simulink library "ConverterLibrary"  (R2026a)
settings: Solver=VariableStepAuto
undefined symbols (not defined in the file or in its folder): DiscIntNeverNeededParam, dspblkCoreblockFVToolHelper, gcbh, gridInverter
libraries: fl_lib x240, nesl_utility x221, ee_lib x208, slpidlib x28, eeGeneralControl x12, simulink x9, eeTransforms x4, simulink_extras x1, eePowerMeasurement x1
(part 9 of 30)

== system ConverterLibrary/Power Converter Plant/Non-Isolated DC-DC Converters/Non-Isolated DC-DC Converter/NonIsolatedDCDCVariant/Boost ==
  G : Inport
  Co : ee_lib/Passive/Capacitor  cap_option=ee.enum.passive.capacitor.capOption.const  c=C_SI F  Cvec=[1e-05, 1e-06] F  Vvec=[0, 10] V  CV_table_symmetry=ee.enum.passive.capacitor.tableSymmetry.yes  f_vec=[1, 10] kHz  DFext_vec=[.8, 1.2]  enable_C_tol=ee.enum.toleranceApplication.none  averaging_period=0 s  C_tol=5  tol_distribution=ee.enum.toleranceDistribution.uniform  nSigma=4  r=Rco_SI Ohm  g=1e-05 1/Ohm  enable_operating_limits=ee.enum.enable.no  operating_limit_action=ee.enum.passive.reportOpLim.warn  max_working_voltage_range=[-25, 25] V  power_rating=1 W  maxTemperature=85 degC  thermalEnable=false  thermalMass=1 J/K  i_specify=off  i_priority=None  i=0 A  i_nominal_specify=off  i_nominal_value=1  i_nominal_unit=A  v_specify=off  v_priority=None  v=0 V  v_nominal_specify=off  v_nominal_value=1  v_nominal_unit=V  vc_specify=on  vc_priority=High  vc=Vco_SI V  vc_nominal_specify=off  vc_nominal_value=1  vc_nominal_unit=V  T_specify=off  T_priority=None  T=298.15 K  T_nominal_specify=off  T_nominal_value=1  T_nominal_unit=K
  Diode : Subsystem  Variant=on  VariantControlMode=label  LabelModeActiveChoice=IdealDiode
  IL : Subsystem
      mask Display: disp('I')
  Iout : Subsystem
      mask Display: disp('I')
  Lin : ee_lib/Passive/Inductor  l=L_SI H  enable_L_tol=ee.enum.toleranceApplication.none  L_tol=20  tol_distribution=ee.enum.toleranceDistribution.uniform  nSigma=4  r=RL_SI Ohm  g=1e-05 1/Ohm  enable_operating_limits=ee.enum.enable.no  operating_limit_action=ee.enum.passive.reportOpLim.warn  max_working_current=1 A  power_rating=1 W  i_L_specify=off  i_L_priority=High  i_L=0 A  i_L_nominal_specify=off  i_L_nominal_value=1  i_L_nominal_unit=A
  MainSwitch : Subsystem  Variant=on  VariantControlMode=label  LabelModeActiveChoice=IdealSwitch
  Vin : Subsystem
      mask Display: disp('V')
  Vout : Subsystem
      settings: PortSchema="{\"entries\":[{\"content\":{\"sides\":[{\"content\":{\"connectorIds\":[\"LConn1\"]},\"type\":\"ConnectorPlacement.EquallySpacedRectSide\",\"uuid\":\"5f92137b-4b58-46b8-a68f-d3527484291c\"},{\"content\":{\"connectorIds\":[\"RConn1\",\"Out1\"],\"side\":\"RIGHT\"},\"type\":\"ConnectorPlacement.EquallySpacedRectSide\",\"uuid\":\"154b36f0-aa4a-4375-80c2-9c55af429c32\"},{\"content\":{\"side\":\"TOP\"},\"type\":\"ConnectorPlacement.EquallySpacedRectSide\",\"uuid\":\"6e01dd2b-817e-4c7e-a9bf-e017a248a3a8\"}]},\"type\":\"ConnectorPlacement.EquallySpacedConnector\",\"uuid\":\"a9d15cc4-68aa-466b-9599-7a273210f999\"}],\"packageUris\":[\"http://schema.mathworks.com/mf0/Connector/R2020b\"],\"version\":\"1.0\"}"
      mask Display: disp('V')
  Vin+ : PMIOPort  Side=Left
  Vin- : PMIOPort  Port=2  Side=Left
  Vout+ : PMIOPort  Port=3  Side=Right
  Vout- : PMIOPort  Port=4  Side=Right
  Out Bus Element1 : Outport  PortName=meas  Element=IL [A]
  Out Bus Element2 : Outport  PortName=meas  Element=Vout [V]
  Out Bus Element3 : Outport  PortName=meas  Element=Iin [A]
  Out Bus Element4 : Outport  PortName=meas  Element=Vin [V]
  Out Bus Element5 : Outport  PortName=meas  Element=Iout [A]
  wires:
  G/1 -> MainSwitch/1(G)
  Iout/1(I) -> Out Bus Element5/1
  Vin/1(V) -> Out Bus Element4/1
  IL/1(I) -> Out Bus Element3/1, Out Bus Element1/1
  Vout/1(V) -> Out Bus Element2/1
  connections:
  Iout/LConn1 -- Co/LConn1 -- Diode/RConn1
  Diode/LConn1 -- MainSwitch/LConn1 -- Lin/RConn1
  Vin/RConn1 -- Vin-/RConn1 -- Vout/RConn1 -- Vout-/RConn1 -- Co/RConn1 -- MainSwitch/RConn1
  Vout/LConn1 -- Iout/RConn1 -- Vout+/RConn1
  IL/RConn1 -- Lin/LConn1
  IL/LConn1 -- Vin/LConn1 -- Vin+/RConn1

== system ConverterLibrary/Power Converter Plant/Non-Isolated DC-DC Converters/Non-Isolated DC-DC Converter/NonIsolatedDCDCVariant/Buck ==
  G : Inport
  Co : ee_lib/Passive/Capacitor  cap_option=ee.enum.passive.capacitor.capOption.const  c=C_SI F  Cvec=[1e-05, 1e-06] F  Vvec=[0, 10] V  CV_table_symmetry=ee.enum.passive.capacitor.tableSymmetry.yes  f_vec=[1, 10] kHz  DFext_vec=[.8, 1.2]  enable_C_tol=ee.enum.toleranceApplication.none  averaging_period=0 s  C_tol=5  tol_distribution=ee.enum.toleranceDistribution.uniform  nSigma=4  r=Rco_SI Ohm  g=1e-05 1/Ohm  enable_operating_limits=ee.enum.enable.no  operating_limit_action=ee.enum.passive.reportOpLim.warn  max_working_voltage_range=[-25, 25] V  power_rating=1 W  maxTemperature=85 degC  thermalEnable=false  thermalMass=1 J/K  i_specify=off  i_priority=None  i=0 A  i_nominal_specify=off  i_nominal_value=1  i_nominal_unit=A  v_specify=off  v_priority=None  v=0 V  v_nominal_specify=off  v_nominal_value=1  v_nominal_unit=V  vc_specify=on  vc_priority=High  vc=Vco_SI V  vc_nominal_specify=off  vc_nominal_value=1  vc_nominal_unit=V  T_specify=off  T_priority=None  T=298.15 K  T_nominal_specify=off  T_nominal_value=1  T_nominal_unit=K
  Diode : Subsystem  Variant=on  VariantControlMode=label  LabelModeActiveChoice=IdealDiode
  IL : Subsystem
      mask Display: disp('I')
  Iin : Subsystem
      mask Display: disp('I')
  Iout : Subsystem
      mask Display: disp('I')
  Lout : ee_lib/Passive/Inductor  l=L_SI H  enable_L_tol=ee.enum.toleranceApplication.none  L_tol=20  tol_distribution=ee.enum.toleranceDistribution.uniform  nSigma=4  r=RL_SI Ohm  g=1e-05 1/Ohm  enable_operating_limits=ee.enum.enable.no  operating_limit_action=ee.enum.passive.reportOpLim.warn  max_working_current=1 A  power_rating=1 W  i_L_specify=off  i_L_priority=High  i_L=0 A  i_L_nominal_specify=off  i_L_nominal_value=1  i_L_nominal_unit=A
  MainSwitch : Subsystem  Variant=on  VariantControlMode=label  LabelModeActiveChoice=IdealSwitch
  Vin : Subsystem
      mask Display: disp('V')
  Vout : Subsystem
      settings: PortSchema="{\"entries\":[{\"content\":{\"sides\":[{\"content\":{\"connectorIds\":[\"LConn1\"]},\"type\":\"ConnectorPlacement.EquallySpacedRectSide\",\"uuid\":\"5f92137b-4b58-46b8-a68f-d3527484291c\"},{\"content\":{\"connectorIds\":[\"RConn1\",\"Out1\"],\"side\":\"RIGHT\"},\"type\":\"ConnectorPlacement.EquallySpacedRectSide\",\"uuid\":\"154b36f0-aa4a-4375-80c2-9c55af429c32\"},{\"content\":{\"side\":\"TOP\"},\"type\":\"ConnectorPlacement.EquallySpacedRectSide\",\"uuid\":\"6e01dd2b-817e-4c7e-a9bf-e017a248a3a8\"}]},\"type\":\"ConnectorPlacement.EquallySpacedConnector\",\"uuid\":\"a9d15cc4-68aa-466b-9599-7a273210f999\"}],\"packageUris\":[\"http://schema.mathworks.com/mf0/Connector/R2020b\"],\"version\":\"1.0\"}"
      mask Display: disp('V')
  Vin+ : PMIOPort  Side=Left
  Vin- : PMIOPort  Port=2  Side=Left
  Vout+ : PMIOPort  Port=3  Side=Right
  Vout- : PMIOPort  Port=4  Side=Right
  Out Bus Element1 : Outport  PortName=meas  Element=IL [A]
  Out Bus Element2 : Outport  PortName=meas  Element=Vout [V]
  Out Bus Element3 : Outport  PortName=meas  Element=Iin [A]
  Out Bus Element4 : Outport  PortName=meas  Element=Vin [V]
  Out Bus Element5 : Outport  PortName=meas  Element=Iout [A]
  wires:
  G/1 -> MainSwitch/1(G)
  Iout/1(I) -> Out Bus Element5/1
  Vin/1(V) -> Out Bus Element4/1
  Iin/1(I) -> Out Bus Element3/1
  Vout/1(V) -> Out Bus Element2/1
  IL/1(I) -> Out Bus Element1/1
  connections:
  Co/RConn1 -- Diode/LConn1 -- Vin/RConn1 -- Vin-/RConn1 -- Vout/RConn1 -- Vout-/RConn1
  Vout/LConn1 -- Vout+/RConn1 -- Iout/RConn1
  Co/LConn1 -- Iout/LConn1 -- IL/RConn1
  Lout/RConn1 -- IL/LConn1
  MainSwitch/RConn1 -- Lout/LConn1 -- Diode/RConn1
  Iin/RConn1 -- MainSwitch/LConn1
  Vin/LConn1 -- Vin+/RConn1 -- Iin/LConn1

== system ConverterLibrary/Power Converter Plant/Non-Isolated DC-DC Converters/Non-Isolated DC-DC Converter/NonIsolatedDCDCVariant/BuckBoost ==
  G : Inport
  Co : ee_lib/Passive/Capacitor  cap_option=ee.enum.passive.capacitor.capOption.const  c=C_SI F  Cvec=[1e-05, 1e-06] F  Vvec=[0, 10] V  CV_table_symmetry=ee.enum.passive.capacitor.tableSymmetry.yes  f_vec=[1, 10] kHz  DFext_vec=[.8, 1.2]  enable_C_tol=ee.enum.toleranceApplication.none  averaging_period=0 s  C_tol=5  tol_distribution=ee.enum.toleranceDistribution.uniform  nSigma=4  r=Rco_SI Ohm  g=1e-05 1/Ohm  enable_operating_limits=ee.enum.enable.no  operating_limit_action=ee.enum.passive.reportOpLim.warn  max_working_voltage_range=[-25, 25] V  power_rating=1 W  maxTemperature=85 degC  thermalEnable=false  thermalMass=1 J/K  i_specify=off  i_priority=None  i=0 A  i_nominal_specify=off  i_nominal_value=1  i_nominal_unit=A  v_specify=off  v_priority=None  v=0 V  v_nominal_specify=off  v_nominal_value=1  v_nominal_unit=V  vc_specify=on  vc_priority=High  vc=Vco_SI V  vc_nominal_specify=off  vc_nominal_value=1  vc_nominal_unit=V  T_specify=off  T_priority=None  T=298.15 K  T_nominal_specify=off  T_nominal_value=1  T_nominal_unit=K
  Diode : Subsystem  Variant=on  VariantControlMode=label  LabelModeActiveChoice=IdealDiode
  IL : Subsystem
      settings: PortSchema="{\"entries\":[{\"content\":{\"sides\":[{\"content\":{\"connectorIds\":[\"LConn1\"]},\"type\":\"ConnectorPlacement.EquallySpacedRectSide\",\"uuid\":\"5f92137b-4b58-46b8-a68f-d3527484291c\"},{\"content\":{\"connectorIds\":[\"RConn1\",\"Out1\"],\"side\":\"RIGHT\"},\"type\":\"ConnectorPlacement.EquallySpacedRectSide\",\"uuid\":\"154b36f0-aa4a-4375-80c2-9c55af429c32\"},{\"content\":{\"side\":\"TOP\"},\"type\":\"ConnectorPlacement.EquallySpacedRectSide\",\"uuid\":\"6e01dd2b-817e-4c7e-a9bf-e017a248a3a8\"},{\"content\":{\"side\":\"BOTTOM\"},\"type\":\"ConnectorPlacement.EquallySpacedRectSide\",\"uuid\":\"8c02900b-7040-4e1d-af3e-df4ce1eee484\"}]},\"type\":\"ConnectorPlacement.EquallySpacedConnector\",\"uuid\":\"a9d15cc4-68aa-466b-9599-7a273210f999\"}],\"packageUris\":[\"http://schema.mathworks.com/mf0/Connector/R2020b\"],\"version\":\"1.0\"}"
      mask Display: disp('I')
  Iin : Subsystem
      mask Display: disp('I')
  Iout : Subsystem
      settings: PortSchema="{\"entries\":[{\"content\":{\"sides\":[{\"content\":{\"connectorIds\":[\"LConn1\"]},\"type\":\"ConnectorPlacement.EquallySpacedRectSide\",\"uuid\":\"7ec392cc-277f-44b1-b35e-7f2730db0397\"},{\"content\":{\"connectorIds\":[\"RConn1\",\"Out1\"],\"side\":\"RIGHT\"},\"type\":\"ConnectorPlacement.EquallySpacedRectSide\",\"uuid\":\"b0b5f2e0-1c59-4384-a465-885626d66149\"},{\"content\":{\"side\":\"TOP\"},\"type\":\"ConnectorPlacement.EquallySpacedRectSide\",\"uuid\":\"04ca4100-95ca-4157-98b9-4ff919847b2d\"}]},\"type\":\"ConnectorPlacement.EquallySpacedConnector\",\"uuid\":\"4f5cd1ed-b6ae-4123-b76e-0cf834717a23\"}],\"packageUris\":[\"http://schema.mathworks.com/mf0/Connector/R2020b\"],\"version\":\"1.0\"}"
      mask Display: disp('I')
  Lstore : ee_lib/Passive/Inductor  l=L_SI H  enable_L_tol=ee.enum.toleranceApplication.none  L_tol=20  tol_distribution=ee.enum.toleranceDistribution.uniform  nSigma=4  r=RL_SI Ohm  g=1e-05 1/Ohm  enable_operating_limits=ee.enum.enable.no  operating_limit_action=ee.enum.passive.reportOpLim.warn  max_working_current=1 A  power_rating=1 W  i_L_specify=off  i_L_priority=High  i_L=0 A  i_L_nominal_specify=off  i_L_nominal_value=1  i_L_nominal_unit=A
  MainSwitch : Subsystem  Variant=on  VariantControlMode=label  LabelModeActiveChoice=IdealSwitch
  Vin : Subsystem
      mask Display: disp('V')
  Vout : Subsystem
      settings: PortSchema="{\"entries\":[{\"content\":{\"sides\":[{\"content\":{\"connectorIds\":[\"LConn1\"]},\"type\":\"ConnectorPlacement.EquallySpacedRectSide\",\"uuid\":\"5f92137b-4b58-46b8-a68f-d3527484291c\"},{\"content\":{\"connectorIds\":[\"RConn1\",\"Out1\"],\"side\":\"RIGHT\"},\"type\":\"ConnectorPlacement.EquallySpacedRectSide\",\"uuid\":\"154b36f0-aa4a-4375-80c2-9c55af429c32\"},{\"content\":{\"side\":\"TOP\"},\"type\":\"ConnectorPlacement.EquallySpacedRectSide\",\"uuid\":\"6e01dd2b-817e-4c7e-a9bf-e017a248a3a8\"}]},\"type\":\"ConnectorPlacement.EquallySpacedConnector\",\"uuid\":\"a9d15cc4-68aa-466b-9599-7a273210f999\"}],\"packageUris\":[\"http://schema.mathworks.com/mf0/Connector/R2020b\"],\"version\":\"1.0\"}"
      mask Display: disp('V')
  Vin+ : PMIOPort  Side=Left
  Vin- : PMIOPort  Port=2  Side=Left
  Vout+ : PMIOPort  Port=3  Side=Right
  Vout- : PMIOPort  Port=4  Side=Right
  Out Bus Element1 : Outport  PortName=meas  Element=IL [A]
  Out Bus Element2 : Outport  PortName=meas  Element=Vout [V]
  Out Bus Element3 : Outport  PortName=meas  Element=Iin [A]
  Out Bus Element4 : Outport  PortName=meas  Element=Vin [V]
  Out Bus Element5 : Outport  PortName=meas  Element=Iout [A]
  wires:
  G/1 -> MainSwitch/1(G)
  Vout/1(V) -> Out Bus Element2/1
  Vin/1(V) -> Out Bus Element4/1
  Iout/1(I) -> Out Bus Element5/1
  Iin/1(I) -> Out Bus Element3/1
  IL/1(I) -> Out Bus Element1/1
  connections:
  Diode/LConn1 -- Vout-/RConn1 -- Vout/RConn1 -- Co/LConn1
  Lstore/LConn1 -- IL/RConn1
  IL/LConn1 -- Diode/RConn1 -- MainSwitch/RConn1
  Lstore/RConn1 -- Co/RConn1 -- Iout/LConn1 -- Vin-/RConn1 -- Vin/RConn1
  Iin/RConn1 -- MainSwitch/LConn1
  Vin/LConn1 -- Vin+/RConn1 -- Iin/LConn1
  Vout+/RConn1 -- Vout/LConn1 -- Iout/RConn1

== system ConverterLibrary/Power Converter Plant/Non-Isolated DC-DC Converters/Non-Isolated DC-DC Converter/NonIsolatedDCDCVariant/SynchronousBoost ==
  G : Inport
  Co : ee_lib/Passive/Capacitor  cap_option=ee.enum.passive.capacitor.capOption.const  c=C_SI F  Cvec=[1e-05, 1e-06] F  Vvec=[0, 10] V  CV_table_symmetry=ee.enum.passive.capacitor.tableSymmetry.yes  f_vec=[1, 10] kHz  DFext_vec=[.8, 1.2]  enable_C_tol=ee.enum.toleranceApplication.none  averaging_period=0 s  C_tol=5  tol_distribution=ee.enum.toleranceDistribution.uniform  nSigma=4  r=Rco_SI Ohm  g=1e-05 1/Ohm  enable_operating_limits=ee.enum.enable.no  operating_limit_action=ee.enum.passive.reportOpLim.warn  max_working_voltage_range=[-25, 25] V  power_rating=1 W  maxTemperature=85 degC  thermalEnable=false  thermalMass=1 J/K  i_specify=off  i_priority=None  i=0 A  i_nominal_specify=off  i_nominal_value=1  i_nominal_unit=A  v_specify=off  v_priority=None  v=0 V  v_nominal_specify=off  v_nominal_value=1  v_nominal_unit=V  vc_specify=on  vc_priority=High  vc=Vco_SI V  vc_nominal_specify=off  vc_nominal_value=1  vc_nominal_unit=V  T_specify=off  T_priority=None  T=298.15 K  T_nominal_specify=off  T_nominal_value=1  T_nominal_unit=K
  Demux : Demux  Outputs=2
  IL : Subsystem
      mask Display: disp('I')
  Iout : Subsystem
      mask Display: disp('I')
  Lin : ee_lib/Passive/Inductor  l=L_SI H  enable_L_tol=ee.enum.toleranceApplication.none  L_tol=20  tol_distribution=ee.enum.toleranceDistribution.uniform  nSigma=4  r=RL_SI Ohm  g=1e-05 1/Ohm  enable_operating_limits=ee.enum.enable.no  operating_limit_action=ee.enum.passive.reportOpLim.warn  max_working_current=1 A  power_rating=1 W  i_L_specify=off  i_L_priority=High  i_L=0 A  i_L_nominal_specify=off  i_L_nominal_value=1  i_L_nominal_unit=A
  MainSwitch : Subsystem  Variant=on  VariantControlMode=label  LabelModeActiveChoice=IdealSwitch
  SyncSwitch : Subsystem  Variant=on  VariantControlMode=label  LabelModeActiveChoice=IdealSwitch
  Vin : Subsystem
      mask Display: disp('V')
  Vout : Subsystem
      settings: PortSchema="{\"entries\":[{\"content\":{\"sides\":[{\"content\":{\"connectorIds\":[\"LConn1\"]},\"type\":\"ConnectorPlacement.EquallySpacedRectSide\",\"uuid\":\"5f92137b-4b58-46b8-a68f-d3527484291c\"},{\"content\":{\"connectorIds\":[\"RConn1\",\"Out1\"],\"side\":\"RIGHT\"},\"type\":\"ConnectorPlacement.EquallySpacedRectSide\",\"uuid\":\"154b36f0-aa4a-4375-80c2-9c55af429c32\"},{\"content\":{\"side\":\"TOP\"},\"type\":\"ConnectorPlacement.EquallySpacedRectSide\",\"uuid\":\"6e01dd2b-817e-4c7e-a9bf-e017a248a3a8\"}]},\"type\":\"ConnectorPlacement.EquallySpacedConnector\",\"uuid\":\"a9d15cc4-68aa-466b-9599-7a273210f999\"}],\"packageUris\":[\"http://schema.mathworks.com/mf0/Connector/R2020b\"],\"version\":\"1.0\"}"
      mask Display: disp('V')
  Vin+ : PMIOPort  Side=Left
  Vin- : PMIOPort  Port=2  Side=Left
  Vout+ : PMIOPort  Port=3  Side=Right
  Vout- : PMIOPort  Port=4  Side=Right
  Out Bus Element1 : Outport  PortName=meas  Element=IL [A]
  Out Bus Element2 : Outport  PortName=meas  Element=Vout [V]
  Out Bus Element3 : Outport  PortName=meas  Element=Iin [A]
  Out Bus Element4 : Outport  PortName=meas  Element=Vin [V]
  Out Bus Element5 : Outport  PortName=meas  Element=Iout [A]
  wires:
  [G1] -> MainSwitch/1(G)
  G/1 -> Demux/1
  Vout/1(V) -> Out Bus Element2/1
  IL/1(I) -> Out Bus Element1/1, Out Bus Element3/1
  Vin/1(V) -> Out Bus Element4/1
  Iout/1(I) -> Out Bus Element5/1
  Demux/1 -> [G1]
  Demux/2 -> [G2]
  [G2] -> SyncSwitch/1(G)
  connections:
  Co/LConn1 -- Iout/LConn1 -- SyncSwitch/LConn1
  Lin/RConn1 -- MainSwitch/LConn1 -- SyncSwitch/RConn1
  Vin/LConn1 -- IL/LConn1 -- Vin+/RConn1
  IL/RConn1 -- Lin/LConn1
  Vout+/RConn1 -- Vout/LConn1 -- Iout/RConn1
  Vin/RConn1 -- MainSwitch/RConn1 -- Vout/RConn1 -- Vout-/RConn1 -- Co/RConn1 -- Vin-/RConn1

== system ConverterLibrary/Power Converter Plant/Non-Isolated DC-DC Converters/Non-Isolated DC-DC Converter/NonIsolatedDCDCVariant/SynchronousBuck ==
  G : Inport
  Co : ee_lib/Passive/Capacitor  cap_option=ee.enum.passive.capacitor.capOption.const  c=C_SI F  Cvec=[1e-05, 1e-06] F  Vvec=[0, 10] V  CV_table_symmetry=ee.enum.passive.capacitor.tableSymmetry.yes  f_vec=[1, 10] kHz  DFext_vec=[.8, 1.2]  enable_C_tol=ee.enum.toleranceApplication.none  averaging_period=0 s  C_tol=5  tol_distribution=ee.enum.toleranceDistribution.uniform  nSigma=4  r=Rco_SI Ohm  g=1e-05 1/Ohm  enable_operating_limits=ee.enum.enable.no  operating_limit_action=ee.enum.passive.reportOpLim.warn  max_working_voltage_range=[-25, 25] V  power_rating=1 W  maxTemperature=85 degC  thermalEnable=false  thermalMass=1 J/K  i_specify=off  i_priority=None  i=0 A  i_nominal_specify=off  i_nominal_value=1  i_nominal_unit=A  v_specify=off  v_priority=None  v=0 V  v_nominal_specify=off  v_nominal_value=1  v_nominal_unit=V  vc_specify=on  vc_priority=High  vc=Vco_SI V  vc_nominal_specify=off  vc_nominal_value=1  vc_nominal_unit=V  T_specify=off  T_priority=None  T=298.15 K  T_nominal_specify=off  T_nominal_value=1  T_nominal_unit=K
  Demux : Demux  Outputs=2
  IL : Subsystem
      mask Display: disp('I')
  Iin : Subsystem
      mask Display: disp('I')
  Iout : Subsystem
      mask Display: disp('I')
  Lout : ee_lib/Passive/Inductor  l=L_SI H  enable_L_tol=ee.enum.toleranceApplication.none  L_tol=20  tol_distribution=ee.enum.toleranceDistribution.uniform  nSigma=4  r=RL_SI Ohm  g=1e-05 1/Ohm  enable_operating_limits=ee.enum.enable.no  operating_limit_action=ee.enum.passive.reportOpLim.warn  max_working_current=1 A  power_rating=1 W  i_L_specify=off  i_L_priority=High  i_L=0 A  i_L_nominal_specify=off  i_L_nominal_value=1  i_L_nominal_unit=A
  MainSwitch : Subsystem  Variant=on  VariantControlMode=label  LabelModeActiveChoice=IdealSwitch
  SyncSwitch : Subsystem  Variant=on  VariantControlMode=label  LabelModeActiveChoice=IdealSwitch
  Vin : Subsystem
      mask Display: disp('V')
  Vout : Subsystem
      settings: PortSchema="{\"entries\":[{\"content\":{\"sides\":[{\"content\":{\"connectorIds\":[\"LConn1\"]},\"type\":\"ConnectorPlacement.EquallySpacedRectSide\",\"uuid\":\"5f92137b-4b58-46b8-a68f-d3527484291c\"},{\"content\":{\"connectorIds\":[\"RConn1\",\"Out1\"],\"side\":\"RIGHT\"},\"type\":\"ConnectorPlacement.EquallySpacedRectSide\",\"uuid\":\"154b36f0-aa4a-4375-80c2-9c55af429c32\"},{\"content\":{\"side\":\"TOP\"},\"type\":\"ConnectorPlacement.EquallySpacedRectSide\",\"uuid\":\"6e01dd2b-817e-4c7e-a9bf-e017a248a3a8\"}]},\"type\":\"ConnectorPlacement.EquallySpacedConnector\",\"uuid\":\"a9d15cc4-68aa-466b-9599-7a273210f999\"}],\"packageUris\":[\"http://schema.mathworks.com/mf0/Connector/R2020b\"],\"version\":\"1.0\"}"
      mask Display: disp('V')
  Vin+ : PMIOPort  Side=Left
  Vin- : PMIOPort  Port=2  Side=Left
  Vout+ : PMIOPort  Port=3  Side=Right
  Vout- : PMIOPort  Port=4  Side=Right
  Out Bus Element1 : Outport  PortName=meas  Element=IL [A]
  Out Bus Element2 : Outport  PortName=meas  Element=Vout [V]
  Out Bus Element3 : Outport  PortName=meas  Element=Iin [A]
  Out Bus Element4 : Outport  PortName=meas  Element=Vin [V]
  Out Bus Element5 : Outport  PortName=meas  Element=Iout [A]
  wires:
  [G2] -> SyncSwitch/1(G)
  [G1] -> MainSwitch/1(G)
  G/1 -> Demux/1
  IL/1(I) -> Out Bus Element1/1
  Vout/1(V) -> Out Bus Element2/1
  Iin/1(I) -> Out Bus Element3/1
  Vin/1(V) -> Out Bus Element4/1
  Iout/1(I) -> Out Bus Element5/1
  Demux/1 -> [G1]
  Demux/2 -> [G2]
  connections:
  Iin/LConn1 -- Vin+/RConn1 -- Vin/LConn1
  Iin/RConn1 -- MainSwitch/LConn1
  MainSwitch/RConn1 -- SyncSwitch/LConn1 -- Lout/LConn1
  Lout/RConn1 -- IL/LConn1
  Co/LConn1 -- IL/RConn1 -- Iout/LConn1
  Iout/RConn1 -- Vout/LConn1 -- Vout+/RConn1
  Vin-/RConn1 -- Vin/RConn1 -- SyncSwitch/RConn1 -- Vout-/RConn1 -- Vout/RConn1 -- Co/RConn1

== system ConverterLibrary/Power Converter Plant/Non-Isolated DC-DC Converters/Non-Isolated DC-DC Converter/NonIsolatedDCDCVariant/SynchronousBuckBoost ==
  G : Inport
  Co : ee_lib/Passive/Capacitor  cap_option=ee.enum.passive.capacitor.capOption.const  c=C_SI F  Cvec=[1e-05, 1e-06] F  Vvec=[0, 10] V  CV_table_symmetry=ee.enum.passive.capacitor.tableSymmetry.yes  f_vec=[1, 10] kHz  DFext_vec=[.8, 1.2]  enable_C_tol=ee.enum.toleranceApplication.none  averaging_period=0 s  C_tol=5  tol_distribution=ee.enum.toleranceDistribution.uniform  nSigma=4  r=Rco_SI Ohm  g=1e-05 1/Ohm  enable_operating_limits=ee.enum.enable.no  operating_limit_action=ee.enum.passive.reportOpLim.warn  max_working_voltage_range=[-25, 25] V  power_rating=1 W  maxTemperature=85 degC  thermalEnable=false  thermalMass=1 J/K  i_specify=off  i_priority=None  i=0 A  i_nominal_specify=off  i_nominal_value=1  i_nominal_unit=A  v_specify=off  v_priority=None  v=0 V  v_nominal_specify=off  v_nominal_value=1  v_nominal_unit=V  vc_specify=on  vc_priority=High  vc=Vco_SI V  vc_nominal_specify=off  vc_nominal_value=1  vc_nominal_unit=V  T_specify=off  T_priority=None  T=298.15 K  T_nominal_specify=off  T_nominal_value=1  T_nominal_unit=K
  Demux : Demux  Outputs=2
  IL : Subsystem
      settings: PortSchema="{\"entries\":[{\"content\":{\"sides\":[{\"content\":{\"connectorIds\":[\"LConn1\"]},\"type\":\"ConnectorPlacement.EquallySpacedRectSide\",\"uuid\":\"5f92137b-4b58-46b8-a68f-d3527484291c\"},{\"content\":{\"connectorIds\":[\"RConn1\",\"Out1\"],\"side\":\"RIGHT\"},\"type\":\"ConnectorPlacement.EquallySpacedRectSide\",\"uuid\":\"154b36f0-aa4a-4375-80c2-9c55af429c32\"},{\"content\":{\"side\":\"TOP\"},\"type\":\"ConnectorPlacement.EquallySpacedRectSide\",\"uuid\":\"6e01dd2b-817e-4c7e-a9bf-e017a248a3a8\"}]},\"type\":\"ConnectorPlacement.EquallySpacedConnector\",\"uuid\":\"a9d15cc4-68aa-466b-9599-7a273210f999\"}],\"packageUris\":[\"http://schema.mathworks.com/mf0/Connector/R2020b\"],\"version\":\"1.0\"}"
      mask Display: disp('I')
  Iin : Subsystem
      mask Display: disp('I')
  Iout : Subsystem
      mask Display: disp('I')
  Lstore : ee_lib/Passive/Inductor  l=L_SI H  enable_L_tol=ee.enum.toleranceApplication.none  L_tol=20  tol_distribution=ee.enum.toleranceDistribution.uniform  nSigma=4  r=RL_SI Ohm  g=1e-05 1/Ohm  enable_operating_limits=ee.enum.enable.no  operating_limit_action=ee.enum.passive.reportOpLim.warn  max_working_current=1 A  power_rating=1 W  i_L_specify=off  i_L_priority=High  i_L=0 A  i_L_nominal_specify=off  i_L_nominal_value=1  i_L_nominal_unit=A
  MainSwitch : Subsystem  Variant=on  VariantControlMode=label  LabelModeActiveChoice=IdealSwitch
  SyncSwitch : Subsystem  Variant=on  VariantControlMode=label  LabelModeActiveChoice=IdealSwitch
  Vin : Subsystem
      mask Display: disp('V')
  Vout : Subsystem
      settings: PortSchema="{\"entries\":[{\"content\":{\"sides\":[{\"content\":{\"connectorIds\":[\"LConn1\"]},\"type\":\"ConnectorPlacement.EquallySpacedRectSide\",\"uuid\":\"5f92137b-4b58-46b8-a68f-d3527484291c\"},{\"content\":{\"connectorIds\":[\"RConn1\",\"Out1\"],\"side\":\"RIGHT\"},\"type\":\"ConnectorPlacement.EquallySpacedRectSide\",\"uuid\":\"154b36f0-aa4a-4375-80c2-9c55af429c32\"},{\"content\":{\"side\":\"TOP\"},\"type\":\"ConnectorPlacement.EquallySpacedRectSide\",\"uuid\":\"6e01dd2b-817e-4c7e-a9bf-e017a248a3a8\"}]},\"type\":\"ConnectorPlacement.EquallySpacedConnector\",\"uuid\":\"a9d15cc4-68aa-466b-9599-7a273210f999\"}],\"packageUris\":[\"http://schema.mathworks.com/mf0/Connector/R2020b\"],\"version\":\"1.0\"}"
      mask Display: disp('V')
  Vin+ : PMIOPort  Side=Left
  Vin- : PMIOPort  Port=2  Side=Left
  Vout+ : PMIOPort  Port=3  Side=Right
  Vout- : PMIOPort  Port=4  Side=Right
  Out Bus Element1 : Outport  PortName=meas  Element=IL [A]
  Out Bus Element2 : Outport  PortName=meas  Element=Vout [V]
  Out Bus Element3 : Outport  PortName=meas  Element=Iin [A]
  Out Bus Element4 : Outport  PortName=meas  Element=Vin [V]
  Out Bus Element5 : Outport  PortName=meas  Element=Iout [A]
  wires:
  IL/1(I) -> Out Bus Element1/1
  [G2] -> SyncSwitch/1(G)
  [G1] -> MainSwitch/1(G)
  G/1 -> Demux/1
  Demux/1 -> [G1]
  Demux/2 -> [G2]
  Iin/1(I) -> Out Bus Element3/1
  Iout/1(I) -> Out Bus Element5/1
  Vin/1(V) -> Out Bus Element4/1
  Vout/1(V) -> Out Bus Element2/1
  connections:
  Iout/RConn1 -- SyncSwitch/RConn1 -- Co/LConn1
  IL/RConn1 -- Lstore/LConn1
  SyncSwitch/LConn1 -- MainSwitch/RConn1 -- IL/LConn1
  Iin/LConn1 -- Vin+/RConn1 -- Vin/LConn1
  Iin/RConn1 -- MainSwitch/LConn1
  Vout-/RConn1 -- Iout/LConn1 -- Vout/RConn1
  Vin-/RConn1 -- Lstore/RConn1 -- Vout/LConn1 -- Vout+/RConn1 -- Co/RConn1 -- Vin/RConn1

== system ConverterLibrary/Power Converter Plant/Power Factor Correction Converters/Boost PFC Converter/BoostPFCVariant/DetailedModel ==
  G : Inport
  BoostDiode : Subsystem  Variant=on  VariantControlMode=label  LabelModeActiveChoice=TabulatedDiode
  BoostSwitch : Subsystem  Variant=on  VariantControlMode=label  LabelModeActiveChoice=SwitchingMOSFETwithThermal
  Co : ee_lib/Passive/Capacitor  cap_option=ee.enum.passive.capacitor.capOption.const  c=CBoost_SI F  Cvec=[1e-05, 1e-06] F  Vvec=[0, 10] V  CV_table_symmetry=ee.enum.passive.capacitor.tableSymmetry.yes  f_vec=[1, 10] kHz  DFext_vec=[.8, 1.2]  enable_C_tol=ee.enum.toleranceApplication.none  averaging_period=0 s  C_tol=5  tol_distribution=ee.enum.toleranceDistribution.uniform  nSigma=4  r=Rco_SI Ohm  g=1e-05 1/Ohm  enable_operating_limits=ee.enum.enable.no  operating_limit_action=ee.enum.passive.reportOpLim.warn  max_working_voltage_range=[-25, 25] V  power_rating=1 W  maxTemperature=85 degC  thermalEnable=false  thermalMass=1 J/K  i_specify=off  i_priority=None  i=0 A  i_nominal_specify=off  i_nominal_value=1  i_nominal_unit=A  v_specify=off  v_priority=None  v=0 V  v_nominal_specify=off  v_nominal_value=1  v_nominal_unit=V  vc_specify=on  vc_priority=High  vc=Vco_SI V  vc_nominal_specify=off  vc_nominal_value=1  vc_nominal_unit=V  T_specify=off  T_priority=None  T=298.15 K  T_nominal_specify=off  T_nominal_value=1  T_nominal_unit=K
  IL : Subsystem
      settings: PortSchema="{\"entries\":[{\"content\":{\"sides\":[{\"content\":{\"connectorIds\":[\"LConn1\"]},\"type\":\"ConnectorPlacement.EquallySpacedRectSide\",\"uuid\":\"80632e7e-66fe-49c8-894c-61cf7358e53a\"},{\"content\":{\"connectorIds\":[\"RConn1\"],\"side\":\"RIGHT\"},\"type\":\"ConnectorPlacement.EquallySpacedRectSide\",\"uuid\":\"7fb991d4-0257-47fa-8c16-238ff3f2e60c\"},{\"content\":{\"connectorIds\":[\"Out1\"],\"side\":\"TOP\"},\"type\":\"ConnectorPlacement.EquallySpacedRectSide\",\"uuid\":\"a2cf4f5e-7cb3-4577-a513-817a4fd9f07d\"}]},\"type\":\"ConnectorPlacement.EquallySpacedConnector\",\"uuid\":\"e3fac4ca-b917-4eeb-beb4-75837a4782c1\"}],\"packageUris\":[\"http://schema.mathworks.com/mf0/Connector/R2020b\"],\"version\":\"1.0\"}"
      mask Display: disp('I')
  Iin : Subsystem
      settings: PortSchema="{\"entries\":[{\"content\":{\"sides\":[{\"content\":{\"connectorIds\":[\"LConn1\"]},\"type\":\"ConnectorPlacement.EquallySpacedRectSide\",\"uuid\":\"80632e7e-66fe-49c8-894c-61cf7358e53a\"},{\"content\":{\"connectorIds\":[\"RConn1\"],\"side\":\"RIGHT\"},\"type\":\"ConnectorPlacement.EquallySpacedRectSide\",\"uuid\":\"7fb991d4-0257-47fa-8c16-238ff3f2e60c\"},{\"content\":{\"connectorIds\":[\"Out1\"],\"side\":\"TOP\"},\"type\":\"ConnectorPlacement.EquallySpacedRectSide\",\"uuid\":\"a2cf4f5e-7cb3-4577-a513-817a4fd9f07d\"}]},\"type\":\"ConnectorPlacement.EquallySpacedConnector\",\"uuid\":\"e3fac4ca-b917-4eeb-beb4-75837a4782c1\"}],\"packageUris\":[\"http://schema.mathworks.com/mf0/Connector/R2020b\"],\"version\":\"1.0\"}"
      mask Display: disp('I')
  Iout : Subsystem
      mask Display: disp('I')
  Lboost : ee_lib/Passive/Inductor  l=LBoost_SI H  enable_L_tol=ee.enum.toleranceApplication.none  L_tol=20  tol_distribution=ee.enum.toleranceDistribution.uniform  nSigma=4  r=RLboost_SI Ohm  g=1e-05 1/Ohm  enable_operating_limits=ee.enum.enable.no  operating_limit_action=ee.enum.passive.reportOpLim.warn  max_working_current=1 A  power_rating=1 W  i_L_specify=off  i_L_priority=High  i_L=0 A  i_L_nominal_specify=off  i_L_nominal_value=1  i_L_nominal_unit=A
  Pre-Charge Diode : fl_lib/Electrical/Electrical Elements/Diode  Vf=VfPreCharge_SI V  Ron=RdPreCharge_SI Ohm  Goff=GdPreCharge_SI 1/Ohm  i_specify=off  i_priority=None  i=0 A  i_nominal_specify=off  i_nominal_value=1  i_nominal_unit=A  v_specify=off  v_priority=None  v=0 V  v_nominal_specify=off  v_nominal_value=1  v_nominal_unit=V
  Pre-Charge Resistor : fl_lib/Electrical/Electrical Elements/Resistor  R=RPreCharge_SI Ohm  i_specify=off  i_priority=None  i=0 A  i_nominal_specify=off  i_nominal_value=1  i_nominal_unit=A  v_specify=off  v_priority=None  v=0 V  v_nominal_specify=off  v_nominal_value=1  v_nominal_unit=V
  RectifierBridge : Subsystem  Variant=on  VariantControlMode=label  LabelModeActiveChoice=TabulatedDiode
  Vin : Subsystem
      mask Display: disp('V')
  Vout : Subsystem
      settings: PortSchema="{\"entries\":[{\"content\":{\"sides\":[{\"content\":{\"connectorIds\":[\"LConn1\"]},\"type\":\"ConnectorPlacement.EquallySpacedRectSide\",\"uuid\":\"80632e7e-66fe-49c8-894c-61cf7358e53a\"},{\"content\":{\"connectorIds\":[\"RConn1\",\"Out1\"],\"side\":\"RIGHT\"},\"type\":\"ConnectorPlacement.EquallySpacedRectSide\",\"uuid\":\"7fb991d4-0257-47fa-8c16-238ff3f2e60c\"},{\"content\":{\"side\":\"TOP\"},\"type\":\"ConnectorPlacement.EquallySpacedRectSide\",\"uuid\":\"a2cf4f5e-7cb3-4577-a513-817a4fd9f07d\"}]},\"type\":\"ConnectorPlacement.EquallySpacedConnector\",\"uuid\":\"e3fac4ca-b917-4eeb-beb4-75837a4782c1\"}],\"packageUris\":[\"http://schema.mathworks.com/mf0/Connector/R2020b\"],\"version\":\"1.0\"}"
      mask Display: disp('V')
  P : PMIOPort  Side=Left
  N : PMIOPort  Port=2  Side=Left
  + : PMIOPort  Port=3  Side=Right
  - : PMIOPort  Port=4  Side=Right
  Out Bus Element1 : Outport  PortName=meas  Element=Iin [A]
  Out Bus Element2 : Outport  PortName=meas  Element=IL [A]
  Out Bus Element3 : Outport  PortName=meas  Element=Vout [V]
  Out Bus Element4 : Outport  PortName=meas  Element=Iout [A]
  Out Bus Element5 : Outport  PortName=meas  Element=Vin [V]
  wires:
  Vin/1(V) -> Out Bus Element5/1
  Iout/1(I) -> Out Bus Element4/1  "Iout [A]"
  Vout/1(V) -> Out Bus Element3/1
  IL/1(I) -> Out Bus Element2/1  "Iin [A]"
  Iin/1(I) -> Out Bus Element1/1  "Iin [A]"
  G/1 -> BoostSwitch/1(G)
  connections:
  Iin/RConn1 -- RectifierBridge/LConn1
  BoostSwitch/RConn1 -- RectifierBridge/RConn2 -- Vout/RConn1 -- -/RConn1 -- Co/RConn1
  Iout/RConn1 -- Vout/LConn1 -- +/RConn1
  Iout/LConn1 -- Pre-Charge Diode/RConn1 -- Co/LConn1 -- BoostDiode/RConn1
  BoostDiode/LConn1 -- IL/RConn1 -- BoostSwitch/LConn1
  Lboost/RConn1 -- IL/LConn1
  RectifierBridge/RConn1 -- Pre-Charge Resistor/LConn1 -- Lboost/LConn1
  RectifierBridge/LConn2 -- Vin/RConn1 -- N/RConn1
  Vin/LConn1 -- Iin/LConn1 -- P/RConn1
  Pre-Charge Resistor/RConn1 -- Pre-Charge Diode/LConn1

== system ConverterLibrary/Power Converter Plant/Power Factor Correction Converters/Boost PFC Converter/BoostPFCVariant/SimplifiedModel ==
  G : Inport
  BoostSwitch : ee_lib/Semiconductors & Converters/Ideal Semiconductor Switch  port_option=ee.enum.controlport.ps  Ron=RdsOn_SI Ohm  Goff=GdsOff_SI 1/Ohm  Vth=Vth_SI V  diode_param=ee.enum.semiconductors.protectionDiode.external  diode_Vf=0.8 V  diode_Ron=0.001 Ohm  diode_Goff=1e-5 1/Ohm  diode_C=50e-9 F  diode_iRM=-235 A  diode_iF=300 A  diode_idot=-50 A/us  diode_trr_param=ee.enum.converters.diodetrr.trr_factor  diode_trr_factor=3  diode_trr=15 us  diode_Qrr=1500 s*uA
  Co : ee_lib/Passive/Capacitor  cap_option=ee.enum.passive.capacitor.capOption.const  c=CBoost_SI F  Cvec=[1e-05, 1e-06] F  Vvec=[0, 10] V  CV_table_symmetry=ee.enum.passive.capacitor.tableSymmetry.yes  f_vec=[1, 10] kHz  DFext_vec=[.8, 1.2]  enable_C_tol=ee.enum.toleranceApplication.none  averaging_period=0 s  C_tol=5  tol_distribution=ee.enum.toleranceDistribution.uniform  nSigma=4  r=Rco_SI Ohm  g=1e-05 1/Ohm  enable_operating_limits=ee.enum.enable.no  operating_limit_action=ee.enum.passive.reportOpLim.warn  max_working_voltage_range=[-25, 25] V  power_rating=1 W  maxTemperature=85 degC  thermalEnable=false  thermalMass=1 J/K  i_specify=off  i_priority=None  i=0 A  i_nominal_specify=off  i_nominal_value=1  i_nominal_unit=A  v_specify=off  v_priority=None  v=0 V  v_nominal_specify=off  v_nominal_value=1  v_nominal_unit=V  vc_specify=on  vc_priority=High  vc=Vco_SI V  vc_nominal_specify=off  vc_nominal_value=1  vc_nominal_unit=V  T_specify=off  T_priority=None  T=298.15 K  T_nominal_specify=off  T_nominal_value=1  T_nominal_unit=K
  Diode1 : fl_lib/Electrical/Electrical Elements/Diode  Vf=VfDiode_SI V  Ron=RdDiode_SI Ohm  Goff=GdDiode_SI 1/Ohm  i_specify=off  i_priority=None  i=0 A  i_nominal_specify=off  i_nominal_value=1  i_nominal_unit=A  v_specify=off  v_priority=None  v=0 V  v_nominal_specify=off  v_nominal_value=1  v_nominal_unit=V
  Diode{2..5} (4 alike) : fl_lib/Electrical/Electrical Elements/Diode  Vf=VfRect_SI V  Ron=RdRect_SI Ohm  Goff=GdRect_SI 1/Ohm  i_specify=off  i_priority=None  i=0 A  i_nominal_specify=off  i_nominal_value=1  i_nominal_unit=A  v_specify=off  v_priority=None  v=0 V  v_nominal_specify=off  v_nominal_value=1  v_nominal_unit=V
  IL : Subsystem
      mask Display: disp('I')
  Iin : Subsystem
      mask Display: disp('I')
  Iout : Subsystem
      mask Display: disp('I')
  Lboost : ee_lib/Passive/Inductor  l=LBoost_SI H  enable_L_tol=ee.enum.toleranceApplication.none  L_tol=20  tol_distribution=ee.enum.toleranceDistribution.uniform  nSigma=4  r=RLboost_SI Ohm  g=1e-05 1/Ohm  enable_operating_limits=ee.enum.enable.no  operating_limit_action=ee.enum.passive.reportOpLim.warn  max_working_current=1 A  power_rating=1 W  i_L_specify=off  i_L_priority=High  i_L=0 A  i_L_nominal_specify=off  i_L_nominal_value=1  i_L_nominal_unit=A
  Pre-Charge Diode : fl_lib/Electrical/Electrical Elements/Diode  Vf=VfPreCharge_SI V  Ron=RdPreCharge_SI Ohm  Goff=GdPreCharge_SI 1/Ohm  i_specify=off  i_priority=None  i=0 A  i_nominal_specify=off  i_nominal_value=1  i_nominal_unit=A  v_specify=off  v_priority=None  v=0 V  v_nominal_specify=off  v_nominal_value=1  v_nominal_unit=V
  Pre-Charge Resistor : fl_lib/Electrical/Electrical Elements/Resistor  R=RPreCharge_SI Ohm  i_specify=off  i_priority=None  i=0 A  i_nominal_specify=off  i_nominal_value=1  i_nominal_unit=A  v_specify=off  v_priority=None  v=0 V  v_nominal_specify=off  v_nominal_value=1  v_nominal_unit=V
  Simulink-PS Converter : nesl_utility/Simulink-PS Converter  PhysicalDomain=network_engine_domain  SubClassName=ps_input  LeftPortType=input  RightPortType=output  PseudoPeriodic=off  Frequencies=[]  NoiseDistribution=none  NoiseParameters=[]  Unit=1  AffineConversion=off  FilteringAndDerivatives=provide  SimscapeFilterOrder=1  InputFilterTimeConstant=0.001  UdotUserProvided=0
  Vin : Subsystem
      settings: PortSchema="{\"entries\":[{\"content\":{\"sides\":[{\"content\":{\"connectorIds\":[\"LConn1\"]},\"type\":\"ConnectorPlacement.EquallySpacedRectSide\",\"uuid\":\"5f92137b-4b58-46b8-a68f-d3527484291c\"},{\"content\":{\"connectorIds\":[\"RConn1\",\"Out1\"],\"side\":\"RIGHT\"},\"type\":\"ConnectorPlacement.EquallySpacedRectSide\",\"uuid\":\"154b36f0-aa4a-4375-80c2-9c55af429c32\"},{\"content\":{\"side\":\"TOP\"},\"type\":\"ConnectorPlacement.EquallySpacedRectSide\",\"uuid\":\"6e01dd2b-817e-4c7e-a9bf-e017a248a3a8\"}]},\"type\":\"ConnectorPlacement.EquallySpacedConnector\",\"uuid\":\"a9d15cc4-68aa-466b-9599-7a273210f999\"}],\"packageUris\":[\"http://schema.mathworks.com/mf0/Connector/R2020b\"],\"version\":\"1.0\"}"
      mask Display: disp('V')
  Vout : Subsystem
      settings: PortSchema="{\"entries\":[{\"content\":{\"sides\":[{\"content\":{\"connectorIds\":[\"LConn1\"]},\"type\":\"ConnectorPlacement.EquallySpacedRectSide\",\"uuid\":\"5f92137b-4b58-46b8-a68f-d3527484291c\"},{\"content\":{\"connectorIds\":[\"RConn1\",\"Out1\"],\"side\":\"RIGHT\"},\"type\":\"ConnectorPlacement.EquallySpacedRectSide\",\"uuid\":\"154b36f0-aa4a-4375-80c2-9c55af429c32\"},{\"content\":{\"side\":\"TOP\"},\"type\":\"ConnectorPlacement.EquallySpacedRectSide\",\"uuid\":\"6e01dd2b-817e-4c7e-a9bf-e017a248a3a8\"}]},\"type\":\"ConnectorPlacement.EquallySpacedConnector\",\"uuid\":\"a9d15cc4-68aa-466b-9599-7a273210f999\"}],\"packageUris\":[\"http://schema.mathworks.com/mf0/Connector/R2020b\"],\"version\":\"1.0\"}"
      mask Display: disp('V')
  P : PMIOPort  Side=Left
  N : PMIOPort  Port=2  Side=Left
  + : PMIOPort  Port=3  Side=Right
  - : PMIOPort  Port=4  Side=Right
  Out Bus Element1 : Outport  PortName=meas  Element=Iin [A]
  Out Bus Element2 : Outport  PortName=meas  Element=IL [A]
  Out Bus Element3 : Outport  PortName=meas  Element=Vout [V]
  Out Bus Element4 : Outport  PortName=meas  Element=Iout [A]
  Out Bus Element5 : Outport  PortName=meas  Element=Vin [V]
  wires:
  G/1 -> Simulink-PS Converter/1
  Iin/1(I) -> Out Bus Element1/1  "Iin [A]"
  Iout/1(I) -> Out Bus Element4/1
  Vout/1(V) -> Out Bus Element3/1
  IL/1(I) -> Out Bus Element2/1
  Vin/1(V) -> Out Bus Element5/1
  connections:
  +/RConn1 -- Vout/LConn1 -- Iout/RConn1
  IL/LConn1 -- Lboost/RConn1
  Iout/LConn1 -- Pre-Charge Diode/RConn1 -- Co/LConn1 -- Diode1/RConn1
  Simulink-PS Converter/RConn1 -- BoostSwitch/LConn1
  BoostSwitch/RConn1 -- IL/RConn1 -- Diode1/LConn1
  Diode3/LConn1 -- BoostSwitch/RConn2 -- Co/RConn1 -- -/RConn1 -- Vout/RConn1 -- Diode5/LConn1
  N/RConn1 -- Diode5/RConn1 -- Diode4/LConn1 -- Vin/RConn1
  Diode2/LConn1 -- Iin/RConn1 -- Diode3/RConn1
  Diode4/RConn1 -- Pre-Charge Resistor/LConn1 -- Lboost/LConn1 -- Diode2/RConn1
  P/RConn1 -- Vin/LConn1 -- Iin/LConn1
  Pre-Charge Diode/LConn1 -- Pre-Charge Resistor/RConn1

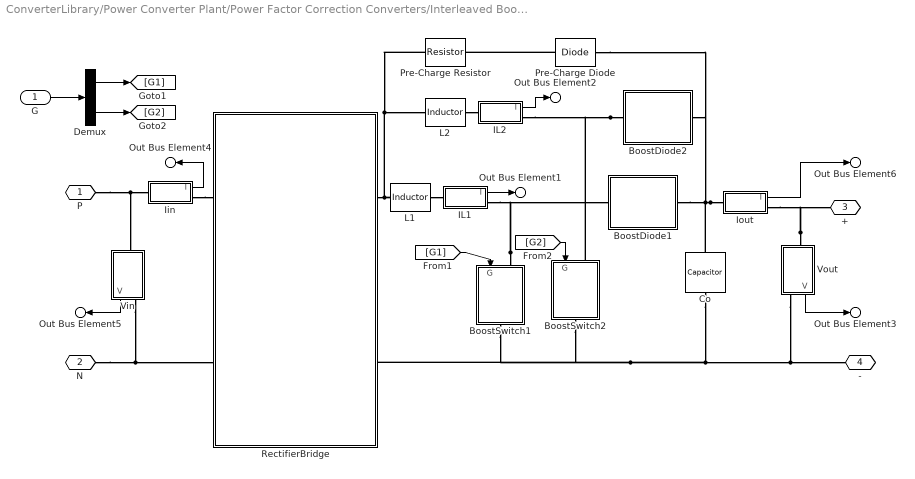
== system ConverterLibrary/Power Converter Plant/Power Factor Correction Converters/Interleaved Boost PFC Converter/InterleavedBoostPFCVariant/DetailedModel ==
  G : Inport
  BoostDiode1 : Subsystem  Variant=on  VariantControlMode=label  LabelModeActiveChoice=TabulatedDiode
  BoostDiode2 : Subsystem  Variant=on  VariantControlMode=label  LabelModeActiveChoice=TabulatedDiode
  BoostSwitch1 : Subsystem  Variant=on  VariantControlMode=label  LabelModeActiveChoice=SwitchingMOSFETwithThermal
  BoostSwitch2 : Subsystem  Variant=on  VariantControlMode=label  LabelModeActiveChoice=SwitchingMOSFETwithThermal
  Co : ee_lib/Passive/Capacitor  cap_option=ee.enum.passive.capacitor.capOption.const  c=CBoost_SI F  Cvec=[1e-05, 1e-06] F  Vvec=[0, 10] V  CV_table_symmetry=ee.enum.passive.capacitor.tableSymmetry.yes  f_vec=[1, 10] kHz  DFext_vec=[.8, 1.2]  enable_C_tol=ee.enum.toleranceApplication.none  averaging_period=0 s  C_tol=5  tol_distribution=ee.enum.toleranceDistribution.uniform  nSigma=4  r=Rco_SI Ohm  g=1e-05 1/Ohm  enable_operating_limits=ee.enum.enable.no  operating_limit_action=ee.enum.passive.reportOpLim.warn  max_working_voltage_range=[-25, 25] V  power_rating=1 W  maxTemperature=85 degC  thermalEnable=false  thermalMass=1 J/K  i_specify=off  i_priority=None  i=0 A  i_nominal_specify=off  i_nominal_value=1  i_nominal_unit=A  v_specify=off  v_priority=None  v=0 V  v_nominal_specify=off  v_nominal_value=1  v_nominal_unit=V  vc_specify=on  vc_priority=High  vc=Vco_SI V  vc_nominal_specify=off  vc_nominal_value=1  vc_nominal_unit=V  T_specify=off  T_priority=None  T=298.15 K  T_nominal_specify=off  T_nominal_value=1  T_nominal_unit=K
  Demux : Demux  Outputs=2
  IL1 : Subsystem
      mask Display: disp('I')
  IL2 : Subsystem
      mask Display: disp('I')
  Iin : Subsystem
      mask Display: disp('I')
  Iout : Subsystem
      mask Display: disp('I')
  L1 : ee_lib/Passive/Inductor  l=LBoost_SI H  enable_L_tol=ee.enum.toleranceApplication.none  L_tol=20  tol_distribution=ee.enum.toleranceDistribution.uniform  nSigma=4  r=RLboost_SI Ohm  g=1e-05 1/Ohm  enable_operating_limits=ee.enum.enable.no  operating_limit_action=ee.enum.passive.reportOpLim.warn  max_working_current=1 A  power_rating=1 W  i_L_specify=off  i_L_priority=High  i_L=0 A  i_L_nominal_specify=off  i_L_nominal_value=1  i_L_nominal_unit=A
  L2 : ee_lib/Passive/Inductor  l=LBoost_SI H  enable_L_tol=ee.enum.toleranceApplication.none  L_tol=20  tol_distribution=ee.enum.toleranceDistribution.uniform  nSigma=4  r=RLboost_SI Ohm  g=1e-05 1/Ohm  enable_operating_limits=ee.enum.enable.no  operating_limit_action=ee.enum.passive.reportOpLim.warn  max_working_current=1 A  power_rating=1 W  i_L_specify=off  i_L_priority=High  i_L=0 A  i_L_nominal_specify=off  i_L_nominal_value=1  i_L_nominal_unit=A
  Pre-Charge Diode : fl_lib/Electrical/Electrical Elements/Diode  Vf=VfPreCharge_SI V  Ron=RdPreCharge_SI Ohm  Goff=GdPreCharge_SI 1/Ohm  i_specify=off  i_priority=None  i=0 A  i_nominal_specify=off  i_nominal_value=1  i_nominal_unit=A  v_specify=off  v_priority=None  v=0 V  v_nominal_specify=off  v_nominal_value=1  v_nominal_unit=V
  Pre-Charge Resistor : fl_lib/Electrical/Electrical Elements/Resistor  R=RPreCharge_SI Ohm  i_specify=off  i_priority=None  i=0 A  i_nominal_specify=off  i_nominal_value=1  i_nominal_unit=A  v_specify=off  v_priority=None  v=0 V  v_nominal_specify=off  v_nominal_value=1  v_nominal_unit=V
  RectifierBridge : Subsystem  Variant=on  VariantControlMode=label  LabelModeActiveChoice=TabulatedDiode
  Vin : Subsystem
      mask Display: disp('V')
  Vout : Subsystem
      settings: PortSchema="{\"entries\":[{\"content\":{\"sides\":[{\"content\":{\"connectorIds\":[\"LConn1\"]},\"type\":\"ConnectorPlacement.EquallySpacedRectSide\",\"uuid\":\"5f92137b-4b58-46b8-a68f-d3527484291c\"},{\"content\":{\"connectorIds\":[\"RConn1\",\"Out1\"],\"side\":\"RIGHT\"},\"type\":\"ConnectorPlacement.EquallySpacedRectSide\",\"uuid\":\"154b36f0-aa4a-4375-80c2-9c55af429c32\"},{\"content\":{\"side\":\"TOP\"},\"type\":\"ConnectorPlacement.EquallySpacedRectSide\",\"uuid\":\"6e01dd2b-817e-4c7e-a9bf-e017a248a3a8\"}]},\"type\":\"ConnectorPlacement.EquallySpacedConnector\",\"uuid\":\"a9d15cc4-68aa-466b-9599-7a273210f999\"}],\"packageUris\":[\"http://schema.mathworks.com/mf0/Connector/R2020b\"],\"version\":\"1.0\"}"
      mask Display: disp('V')
  P : PMIOPort  Side=Left
  N : PMIOPort  Port=2  Side=Left
  + : PMIOPort  Port=3  Side=Right
  - : PMIOPort  Port=4  Side=Right
  Out Bus Element1 : Outport  PortName=meas  Element=IL1 [A]
  Out Bus Element2 : Outport  PortName=meas  Element=IL2 [A]
  Out Bus Element3 : Outport  PortName=meas  Element=Vout [V]
  Out Bus Element4 : Outport  PortName=meas  Element=Iin [A]
  Out Bus Element5 : Outport  PortName=meas  Element=Vin [V]
  Out Bus Element6 : Outport  PortName=meas  Element=Iout [A]
  wires:
  Vout/1(V) -> Out Bus Element3/1
  Vin/1(V) -> Out Bus Element5/1
  Iout/1(I) -> Out Bus Element6/1
  Iin/1(I) -> Out Bus Element4/1
  IL2/1(I) -> Out Bus Element2/1
  IL1/1(I) -> Out Bus Element1/1
  [G2] -> BoostSwitch2/1(G)
  [G1] -> BoostSwitch1/1(G)
  Demux/2 -> [G2]
  Demux/1 -> [G1]
  G/1 -> Demux/1
  connections:
  BoostDiode2/LConn1 -- BoostSwitch2/LConn1 -- IL2/RConn1
  Co/RConn1 -- Vout/RConn1 -- -/RConn1 -- BoostSwitch2/RConn1 -- BoostSwitch1/RConn1 -- RectifierBridge/RConn2
  Vout/LConn1 -- +/RConn1 -- Iout/RConn1
  Iout/LConn1 -- Pre-Charge Diode/RConn1 -- BoostDiode2/RConn1 -- Co/LConn1 -- BoostDiode1/RConn1
  L2/RConn1 -- IL2/LConn1
  BoostSwitch1/LConn1 -- BoostDiode1/LConn1 -- IL1/RConn1
  L1/RConn1 -- IL1/LConn1
  RectifierBridge/RConn1 -- L1/LConn1 -- Pre-Charge Resistor/LConn1 -- L2/LConn1
  Vin/RConn1 -- N/RConn1 -- RectifierBridge/LConn2
  Iin/RConn1 -- RectifierBridge/LConn1
  P/RConn1 -- Vin/LConn1 -- Iin/LConn1
  Pre-Charge Diode/LConn1 -- Pre-Charge Resistor/RConn1
